simulink subsystem "Model_of_Sensors"  (R2025b)
settings: Solver=VariableStepAuto  StartTime=0.0  StopTime=10.0  RelTol=1e-3
settings Model: Creator=Admin  LastModifiedBy=Admin

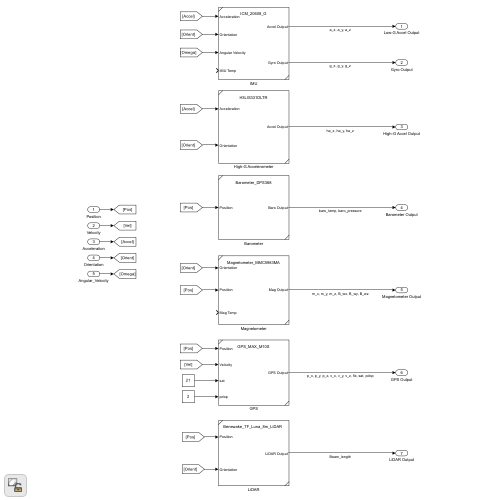
[thumbnail: Simulink's stored preview of the top-level diagram]
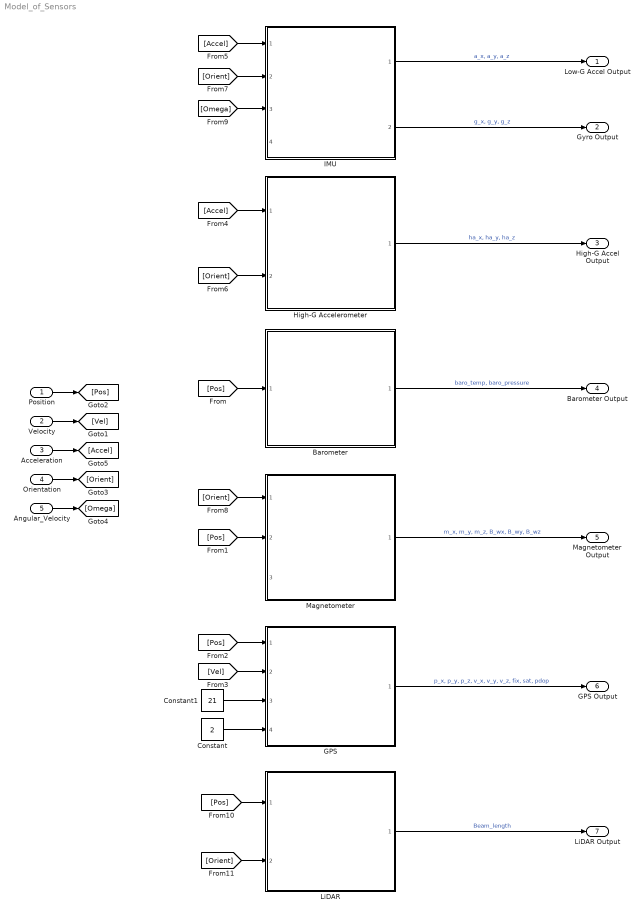
== system Model_of_Sensors ==
  Position : Inport
  Velocity : Inport  Port=2
  Acceleration : Inport  Port=3
  Orientation : Inport  Port=4
  Angular_Velocity : Inport  Port=5
  Barometer : Subsystem  ReferencedSubsystem=Barometer_DPS368
  Constant : Constant  Value=2
  Constant1 : Constant  Value=21
  GPS : Subsystem  ReferencedSubsystem=GPS_MAX_M10S
  "High-G Accelerometer " : Subsystem  ReferencedSubsystem=H3LIS331DLTR
  IMU : Subsystem  ReferencedSubsystem=ICM_20608_G
  LiDAR : Subsystem  ReferencedSubsystem=Benewake_TF_Luna_8m_LiDAR
  Magnetometer : Subsystem  ReferencedSubsystem=Magnetometer_MMC5983MA
  Low-G Accel Output : Outport
  Gyro Output : Outport  Port=2
  High-G Accel Output : Outport  Port=3
  Barometer Output : Outport  Port=4
  Magnetometer Output : Outport  Port=5
  GPS Output : Outport  Port=6
  LiDAR Output : Outport  Port=7
  wires:
  "High-G Accelerometer "/1 -> High-G Accel Output/1  "ha_x, ha_y, ha_z"
  GPS/1 -> GPS Output/1  "p_x, p_y, p_z, v_x, v_y, v_z, fix, sat, pdop"
  Constant/1 -> GPS/4
  Constant1/1 -> GPS/3
  Magnetometer/1 -> Magnetometer Output/1  "m_x, m_y, m_z, B_wx, B_wy, B_wz"
  Position/1 -> [Pos]
  Acceleration/1 -> [Accel]
  Velocity/1 -> [Vel]
  Orientation/1 -> [Orient]
  Angular_Velocity/1 -> [Omega]
  [Pos] -> Magnetometer/2
  [Pos] -> GPS/1
  [Vel] -> GPS/2
  [Accel] -> "High-G Accelerometer "/1
  [Accel] -> IMU/1
  [Orient] -> "High-G Accelerometer "/2
  [Orient] -> IMU/2
  [Orient] -> Magnetometer/1
  [Omega] -> IMU/3
  [Pos] -> LiDAR/1
  [Orient] -> LiDAR/2
  IMU/1 -> Low-G Accel Output/1  "a_x, a_y, a_z"
  IMU/2 -> Gyro Output/1  "g_x, g_y, g_z"
  LiDAR/1 -> LiDAR Output/1  "Beam_length"
  Barometer/1 -> Barometer Output/1  "baro_temp, baro_pressure"
  [Pos] -> Barometer/1
